simulink model "rfsoc4x2_ospfb_128"  (R2021a)
settings: Solver=VariableStepAuto  StartTime=0.0  StopTime=2048  RelTol=1e-3
undefined symbols (not defined in the file): pfb_coeff_gen_calc
libraries: xbsIndex_r4 x25898, casper_library_delays x113, casper_library_misc x68, xps_library x1
(part 49 of 221)

== system rfsoc4x2_ospfb_128/pfb_fir_real7/pol1_in1_first_tap2/delay_bram ==
  din : Inport
  constant : xbsIndex_r4/Constant  const=1  gui_display_data_type=Fixed-point  arith_type=Boolean  n_bits=16  bin_pt=14  preci_type=Single  exp_width=8  frac_width=24  explicit_period=on  period=1  equ=P=C  opselect=C  inp2=PCIN>>17  opr=+  inp1=P  carry=CIN  dbl_ovrd=off  block_type=constant
  counter : xbsIndex_r4/Counter  cnt_type=Count Limited  cnt_to=DelayLen - bram_latency - 1  operation=Up  start_count=0  cnt_by_val=1  arith_type=Unsigned  n_bits=4  bin_pt=0  load_pin=off  rst=off  en=off  explicit_period=on  period=1  use_behavioral_HDL=on  implementation=Fabric  use_rpm=off  dbl_ovrd=off  block_type=counter
  ram : xbsIndex_r4/Single Port RAM  depth=16  initVector=0  distributed_mem=Block RAM  write_mode=Read Before Write  rst=off  init_reg=0  en=off  optimize_latency=off  latency=bram_latency  optimize=Area  dbl_ovrd=off  simulation_type=fast_sim  block_type=spram
  dout : Outport  VectorParamsAs1DForOutWhenUnconnected=off
  wires:
  ram/1 -> dout/1
  constant/1 -> ram/3
  din/1 -> ram/2
  counter/1 -> ram/1

== system rfsoc4x2_ospfb_128/pfb_fir_real7/pol1_in1_first_tap3/delay_bram ==
  din : Inport
  constant : xbsIndex_r4/Constant  const=1  gui_display_data_type=Fixed-point  arith_type=Boolean  n_bits=16  bin_pt=14  preci_type=Single  exp_width=8  frac_width=24  explicit_period=on  period=1  equ=P=C  opselect=C  inp2=PCIN>>17  opr=+  inp1=P  carry=CIN  dbl_ovrd=off  block_type=constant
  counter : xbsIndex_r4/Counter  cnt_type=Count Limited  cnt_to=DelayLen - bram_latency - 1  operation=Up  start_count=0  cnt_by_val=1  arith_type=Unsigned  n_bits=4  bin_pt=0  load_pin=off  rst=off  en=off  explicit_period=on  period=1  use_behavioral_HDL=on  implementation=Fabric  use_rpm=off  dbl_ovrd=off  block_type=counter
  ram : xbsIndex_r4/Single Port RAM  depth=16  initVector=0  distributed_mem=Block RAM  write_mode=Read Before Write  rst=off  init_reg=0  en=off  optimize_latency=off  latency=bram_latency  optimize=Area  dbl_ovrd=off  simulation_type=fast_sim  block_type=spram
  dout : Outport  VectorParamsAs1DForOutWhenUnconnected=off
  wires:
  ram/1 -> dout/1
  constant/1 -> ram/3
  din/1 -> ram/2
  counter/1 -> ram/1

== system rfsoc4x2_ospfb_128/pfb_fir_real7/pol1_in1_first_tap4/delay_bram ==
  din : Inport
  constant : xbsIndex_r4/Constant  const=1  gui_display_data_type=Fixed-point  arith_type=Boolean  n_bits=16  bin_pt=14  preci_type=Single  exp_width=8  frac_width=24  explicit_period=on  period=1  equ=P=C  opselect=C  inp2=PCIN>>17  opr=+  inp1=P  carry=CIN  dbl_ovrd=off  block_type=constant
  counter : xbsIndex_r4/Counter  cnt_type=Count Limited  cnt_to=DelayLen - bram_latency - 1  operation=Up  start_count=0  cnt_by_val=1  arith_type=Unsigned  n_bits=4  bin_pt=0  load_pin=off  rst=off  en=off  explicit_period=on  period=1  use_behavioral_HDL=on  implementation=Fabric  use_rpm=off  dbl_ovrd=off  block_type=counter
  ram : xbsIndex_r4/Single Port RAM  depth=16  initVector=0  distributed_mem=Block RAM  write_mode=Read Before Write  rst=off  init_reg=0  en=off  optimize_latency=off  latency=bram_latency  optimize=Area  dbl_ovrd=off  simulation_type=fast_sim  block_type=spram
  dout : Outport  VectorParamsAs1DForOutWhenUnconnected=off
  wires:
  ram/1 -> dout/1
  constant/1 -> ram/3
  din/1 -> ram/2
  counter/1 -> ram/1

== system rfsoc4x2_ospfb_128/pfb_fir_real7/pol1_in1_first_tap5/delay_bram ==
  din : Inport
  constant : xbsIndex_r4/Constant  const=1  gui_display_data_type=Fixed-point  arith_type=Boolean  n_bits=16  bin_pt=14  preci_type=Single  exp_width=8  frac_width=24  explicit_period=on  period=1  equ=P=C  opselect=C  inp2=PCIN>>17  opr=+  inp1=P  carry=CIN  dbl_ovrd=off  block_type=constant
  counter : xbsIndex_r4/Counter  cnt_type=Count Limited  cnt_to=DelayLen - bram_latency - 1  operation=Up  start_count=0  cnt_by_val=1  arith_type=Unsigned  n_bits=4  bin_pt=0  load_pin=off  rst=off  en=off  explicit_period=on  period=1  use_behavioral_HDL=on  implementation=Fabric  use_rpm=off  dbl_ovrd=off  block_type=counter
  ram : xbsIndex_r4/Single Port RAM  depth=16  initVector=0  distributed_mem=Block RAM  write_mode=Read Before Write  rst=off  init_reg=0  en=off  optimize_latency=off  latency=bram_latency  optimize=Area  dbl_ovrd=off  simulation_type=fast_sim  block_type=spram
  dout : Outport  VectorParamsAs1DForOutWhenUnconnected=off
  wires:
  ram/1 -> dout/1
  constant/1 -> ram/3
  din/1 -> ram/2
  counter/1 -> ram/1

== system rfsoc4x2_ospfb_128/pfb_fir_real7/pol1_in1_first_tap6/delay_bram ==
  din : Inport
  constant : xbsIndex_r4/Constant  const=1  gui_display_data_type=Fixed-point  arith_type=Boolean  n_bits=16  bin_pt=14  preci_type=Single  exp_width=8  frac_width=24  explicit_period=on  period=1  equ=P=C  opselect=C  inp2=PCIN>>17  opr=+  inp1=P  carry=CIN  dbl_ovrd=off  block_type=constant
  counter : xbsIndex_r4/Counter  cnt_type=Count Limited  cnt_to=DelayLen - bram_latency - 1  operation=Up  start_count=0  cnt_by_val=1  arith_type=Unsigned  n_bits=4  bin_pt=0  load_pin=off  rst=off  en=off  explicit_period=on  period=1  use_behavioral_HDL=on  implementation=Fabric  use_rpm=off  dbl_ovrd=off  block_type=counter
  ram : xbsIndex_r4/Single Port RAM  depth=16  initVector=0  distributed_mem=Block RAM  write_mode=Read Before Write  rst=off  init_reg=0  en=off  optimize_latency=off  latency=bram_latency  optimize=Area  dbl_ovrd=off  simulation_type=fast_sim  block_type=spram
  dout : Outport  VectorParamsAs1DForOutWhenUnconnected=off
  wires:
  ram/1 -> dout/1
  constant/1 -> ram/3
  din/1 -> ram/2
  counter/1 -> ram/1

== system rfsoc4x2_ospfb_128/pfb_fir_real7/pol1_in1_first_tap7/delay_bram ==
  din : Inport
  constant : xbsIndex_r4/Constant  const=1  gui_display_data_type=Fixed-point  arith_type=Boolean  n_bits=16  bin_pt=14  preci_type=Single  exp_width=8  frac_width=24  explicit_period=on  period=1  equ=P=C  opselect=C  inp2=PCIN>>17  opr=+  inp1=P  carry=CIN  dbl_ovrd=off  block_type=constant
  counter : xbsIndex_r4/Counter  cnt_type=Count Limited  cnt_to=DelayLen - bram_latency - 1  operation=Up  start_count=0  cnt_by_val=1  arith_type=Unsigned  n_bits=4  bin_pt=0  load_pin=off  rst=off  en=off  explicit_period=on  period=1  use_behavioral_HDL=on  implementation=Fabric  use_rpm=off  dbl_ovrd=off  block_type=counter
  ram : xbsIndex_r4/Single Port RAM  depth=16  initVector=0  distributed_mem=Block RAM  write_mode=Read Before Write  rst=off  init_reg=0  en=off  optimize_latency=off  latency=bram_latency  optimize=Area  dbl_ovrd=off  simulation_type=fast_sim  block_type=spram
  dout : Outport  VectorParamsAs1DForOutWhenUnconnected=off
  wires:
  ram/1 -> dout/1
  constant/1 -> ram/3
  din/1 -> ram/2
  counter/1 -> ram/1

== system rfsoc4x2_ospfb_128/pfb_fir_real7/pol1_in1_first_tap8/delay_bram ==
  din : Inport
  constant : xbsIndex_r4/Constant  const=1  gui_display_data_type=Fixed-point  arith_type=Boolean  n_bits=16  bin_pt=14  preci_type=Single  exp_width=8  frac_width=24  explicit_period=on  period=1  equ=P=C  opselect=C  inp2=PCIN>>17  opr=+  inp1=P  carry=CIN  dbl_ovrd=off  block_type=constant
  counter : xbsIndex_r4/Counter  cnt_type=Count Limited  cnt_to=DelayLen - bram_latency - 1  operation=Up  start_count=0  cnt_by_val=1  arith_type=Unsigned  n_bits=4  bin_pt=0  load_pin=off  rst=off  en=off  explicit_period=on  period=1  use_behavioral_HDL=on  implementation=Fabric  use_rpm=off  dbl_ovrd=off  block_type=counter
  ram : xbsIndex_r4/Single Port RAM  depth=16  initVector=0  distributed_mem=Block RAM  write_mode=Read Before Write  rst=off  init_reg=0  en=off  optimize_latency=off  latency=bram_latency  optimize=Area  dbl_ovrd=off  simulation_type=fast_sim  block_type=spram
  dout : Outport  VectorParamsAs1DForOutWhenUnconnected=off
  wires:
  ram/1 -> dout/1
  constant/1 -> ram/3
  din/1 -> ram/2
  counter/1 -> ram/1

== system rfsoc4x2_ospfb_128/pfb_fir_real7/pol1_in1_first_tap9/delay_bram ==
  din : Inport
  constant : xbsIndex_r4/Constant  const=1  gui_display_data_type=Fixed-point  arith_type=Boolean  n_bits=16  bin_pt=14  preci_type=Single  exp_width=8  frac_width=24  explicit_period=on  period=1  equ=P=C  opselect=C  inp2=PCIN>>17  opr=+  inp1=P  carry=CIN  dbl_ovrd=off  block_type=constant
  counter : xbsIndex_r4/Counter  cnt_type=Count Limited  cnt_to=DelayLen - bram_latency - 1  operation=Up  start_count=0  cnt_by_val=1  arith_type=Unsigned  n_bits=4  bin_pt=0  load_pin=off  rst=off  en=off  explicit_period=on  period=1  use_behavioral_HDL=on  implementation=Fabric  use_rpm=off  dbl_ovrd=off  block_type=counter
  ram : xbsIndex_r4/Single Port RAM  depth=16  initVector=0  distributed_mem=Block RAM  write_mode=Read Before Write  rst=off  init_reg=0  en=off  optimize_latency=off  latency=bram_latency  optimize=Area  dbl_ovrd=off  simulation_type=fast_sim  block_type=spram
  dout : Outport  VectorParamsAs1DForOutWhenUnconnected=off
  wires:
  ram/1 -> dout/1
  constant/1 -> ram/3
  din/1 -> ram/2
  counter/1 -> ram/1

== system rfsoc4x2_ospfb_128/pfb_fir_real7/pol1_in1_tap1/delay_bram ==
  din : Inport
  constant : xbsIndex_r4/Constant  const=1  gui_display_data_type=Fixed-point  arith_type=Boolean  n_bits=16  bin_pt=14  preci_type=Single  exp_width=8  frac_width=24  explicit_period=on  period=1  equ=P=C  opselect=C  inp2=PCIN>>17  opr=+  inp1=P  carry=CIN  dbl_ovrd=off  block_type=constant
  counter : xbsIndex_r4/Counter  cnt_type=Count Limited  cnt_to=DelayLen - bram_latency - 1  operation=Up  start_count=0  cnt_by_val=1  arith_type=Unsigned  n_bits=4  bin_pt=0  load_pin=off  rst=off  en=off  explicit_period=on  period=1  use_behavioral_HDL=on  implementation=Fabric  use_rpm=off  dbl_ovrd=off  block_type=counter
  ram : xbsIndex_r4/Single Port RAM  depth=16  initVector=0  distributed_mem=Block RAM  write_mode=Read Before Write  rst=off  init_reg=0  en=off  optimize_latency=off  latency=bram_latency  optimize=Area  dbl_ovrd=off  simulation_type=fast_sim  block_type=spram
  dout : Outport  VectorParamsAs1DForOutWhenUnconnected=off
  wires:
  ram/1 -> dout/1
  constant/1 -> ram/3
  din/1 -> ram/2
  counter/1 -> ram/1

== system rfsoc4x2_ospfb_128/pfb_fir_real7/pol1_in1_tap10/delay_bram ==
  din : Inport
  constant : xbsIndex_r4/Constant  const=1  gui_display_data_type=Fixed-point  arith_type=Boolean  n_bits=16  bin_pt=14  preci_type=Single  exp_width=8  frac_width=24  explicit_period=on  period=1  equ=P=C  opselect=C  inp2=PCIN>>17  opr=+  inp1=P  carry=CIN  dbl_ovrd=off  block_type=constant
  counter : xbsIndex_r4/Counter  cnt_type=Count Limited  cnt_to=DelayLen - bram_latency - 1  operation=Up  start_count=0  cnt_by_val=1  arith_type=Unsigned  n_bits=4  bin_pt=0  load_pin=off  rst=off  en=off  explicit_period=on  period=1  use_behavioral_HDL=on  implementation=Fabric  use_rpm=off  dbl_ovrd=off  block_type=counter
  ram : xbsIndex_r4/Single Port RAM  depth=16  initVector=0  distributed_mem=Block RAM  write_mode=Read Before Write  rst=off  init_reg=0  en=off  optimize_latency=off  latency=bram_latency  optimize=Area  dbl_ovrd=off  simulation_type=fast_sim  block_type=spram
  dout : Outport  VectorParamsAs1DForOutWhenUnconnected=off
  wires:
  ram/1 -> dout/1
  constant/1 -> ram/3
  din/1 -> ram/2
  counter/1 -> ram/1

== system rfsoc4x2_ospfb_128/pfb_fir_real7/pol1_in1_tap11/delay_bram ==
  din : Inport
  constant : xbsIndex_r4/Constant  const=1  gui_display_data_type=Fixed-point  arith_type=Boolean  n_bits=16  bin_pt=14  preci_type=Single  exp_width=8  frac_width=24  explicit_period=on  period=1  equ=P=C  opselect=C  inp2=PCIN>>17  opr=+  inp1=P  carry=CIN  dbl_ovrd=off  block_type=constant
  counter : xbsIndex_r4/Counter  cnt_type=Count Limited  cnt_to=DelayLen - bram_latency - 1  operation=Up  start_count=0  cnt_by_val=1  arith_type=Unsigned  n_bits=4  bin_pt=0  load_pin=off  rst=off  en=off  explicit_period=on  period=1  use_behavioral_HDL=on  implementation=Fabric  use_rpm=off  dbl_ovrd=off  block_type=counter
  ram : xbsIndex_r4/Single Port RAM  depth=16  initVector=0  distributed_mem=Block RAM  write_mode=Read Before Write  rst=off  init_reg=0  en=off  optimize_latency=off  latency=bram_latency  optimize=Area  dbl_ovrd=off  simulation_type=fast_sim  block_type=spram
  dout : Outport  VectorParamsAs1DForOutWhenUnconnected=off
  wires:
  ram/1 -> dout/1
  constant/1 -> ram/3
  din/1 -> ram/2
  counter/1 -> ram/1

== system rfsoc4x2_ospfb_128/pfb_fir_real7/pol1_in1_tap12/delay_bram ==
  din : Inport
  constant : xbsIndex_r4/Constant  const=1  gui_display_data_type=Fixed-point  arith_type=Boolean  n_bits=16  bin_pt=14  preci_type=Single  exp_width=8  frac_width=24  explicit_period=on  period=1  equ=P=C  opselect=C  inp2=PCIN>>17  opr=+  inp1=P  carry=CIN  dbl_ovrd=off  block_type=constant
  counter : xbsIndex_r4/Counter  cnt_type=Count Limited  cnt_to=DelayLen - bram_latency - 1  operation=Up  start_count=0  cnt_by_val=1  arith_type=Unsigned  n_bits=4  bin_pt=0  load_pin=off  rst=off  en=off  explicit_period=on  period=1  use_behavioral_HDL=on  implementation=Fabric  use_rpm=off  dbl_ovrd=off  block_type=counter
  ram : xbsIndex_r4/Single Port RAM  depth=16  initVector=0  distributed_mem=Block RAM  write_mode=Read Before Write  rst=off  init_reg=0  en=off  optimize_latency=off  latency=bram_latency  optimize=Area  dbl_ovrd=off  simulation_type=fast_sim  block_type=spram
  dout : Outport  VectorParamsAs1DForOutWhenUnconnected=off
  wires:
  ram/1 -> dout/1
  constant/1 -> ram/3
  din/1 -> ram/2
  counter/1 -> ram/1

== system rfsoc4x2_ospfb_128/pfb_fir_real7/pol1_in1_tap13/delay_bram ==
  din : Inport
  constant : xbsIndex_r4/Constant  const=1  gui_display_data_type=Fixed-point  arith_type=Boolean  n_bits=16  bin_pt=14  preci_type=Single  exp_width=8  frac_width=24  explicit_period=on  period=1  equ=P=C  opselect=C  inp2=PCIN>>17  opr=+  inp1=P  carry=CIN  dbl_ovrd=off  block_type=constant
  counter : xbsIndex_r4/Counter  cnt_type=Count Limited  cnt_to=DelayLen - bram_latency - 1  operation=Up  start_count=0  cnt_by_val=1  arith_type=Unsigned  n_bits=4  bin_pt=0  load_pin=off  rst=off  en=off  explicit_period=on  period=1  use_behavioral_HDL=on  implementation=Fabric  use_rpm=off  dbl_ovrd=off  block_type=counter
  ram : xbsIndex_r4/Single Port RAM  depth=16  initVector=0  distributed_mem=Block RAM  write_mode=Read Before Write  rst=off  init_reg=0  en=off  optimize_latency=off  latency=bram_latency  optimize=Area  dbl_ovrd=off  simulation_type=fast_sim  block_type=spram
  dout : Outport  VectorParamsAs1DForOutWhenUnconnected=off
  wires:
  ram/1 -> dout/1
  constant/1 -> ram/3
  din/1 -> ram/2
  counter/1 -> ram/1

== system rfsoc4x2_ospfb_128/pfb_fir_real7/pol1_in1_tap14/delay_bram ==
  din : Inport
  constant : xbsIndex_r4/Constant  const=1  gui_display_data_type=Fixed-point  arith_type=Boolean  n_bits=16  bin_pt=14  preci_type=Single  exp_width=8  frac_width=24  explicit_period=on  period=1  equ=P=C  opselect=C  inp2=PCIN>>17  opr=+  inp1=P  carry=CIN  dbl_ovrd=off  block_type=constant
  counter : xbsIndex_r4/Counter  cnt_type=Count Limited  cnt_to=DelayLen - bram_latency - 1  operation=Up  start_count=0  cnt_by_val=1  arith_type=Unsigned  n_bits=4  bin_pt=0  load_pin=off  rst=off  en=off  explicit_period=on  period=1  use_behavioral_HDL=on  implementation=Fabric  use_rpm=off  dbl_ovrd=off  block_type=counter
  ram : xbsIndex_r4/Single Port RAM  depth=16  initVector=0  distributed_mem=Block RAM  write_mode=Read Before Write  rst=off  init_reg=0  en=off  optimize_latency=off  latency=bram_latency  optimize=Area  dbl_ovrd=off  simulation_type=fast_sim  block_type=spram
  dout : Outport  VectorParamsAs1DForOutWhenUnconnected=off
  wires:
  ram/1 -> dout/1
  constant/1 -> ram/3
  din/1 -> ram/2
  counter/1 -> ram/1

== system rfsoc4x2_ospfb_128/pfb_fir_real7/pol1_in1_tap15/delay_bram ==
  din : Inport
  constant : xbsIndex_r4/Constant  const=1  gui_display_data_type=Fixed-point  arith_type=Boolean  n_bits=16  bin_pt=14  preci_type=Single  exp_width=8  frac_width=24  explicit_period=on  period=1  equ=P=C  opselect=C  inp2=PCIN>>17  opr=+  inp1=P  carry=CIN  dbl_ovrd=off  block_type=constant
  counter : xbsIndex_r4/Counter  cnt_type=Count Limited  cnt_to=DelayLen - bram_latency - 1  operation=Up  start_count=0  cnt_by_val=1  arith_type=Unsigned  n_bits=4  bin_pt=0  load_pin=off  rst=off  en=off  explicit_period=on  period=1  use_behavioral_HDL=on  implementation=Fabric  use_rpm=off  dbl_ovrd=off  block_type=counter
  ram : xbsIndex_r4/Single Port RAM  depth=16  initVector=0  distributed_mem=Block RAM  write_mode=Read Before Write  rst=off  init_reg=0  en=off  optimize_latency=off  latency=bram_latency  optimize=Area  dbl_ovrd=off  simulation_type=fast_sim  block_type=spram
  dout : Outport  VectorParamsAs1DForOutWhenUnconnected=off
  wires:
  ram/1 -> dout/1
  constant/1 -> ram/3
  din/1 -> ram/2
  counter/1 -> ram/1

== system rfsoc4x2_ospfb_128/pfb_fir_real7/pol1_in1_tap16/delay_bram ==
  din : Inport
  constant : xbsIndex_r4/Constant  const=1  gui_display_data_type=Fixed-point  arith_type=Boolean  n_bits=16  bin_pt=14  preci_type=Single  exp_width=8  frac_width=24  explicit_period=on  period=1  equ=P=C  opselect=C  inp2=PCIN>>17  opr=+  inp1=P  carry=CIN  dbl_ovrd=off  block_type=constant
  counter : xbsIndex_r4/Counter  cnt_type=Count Limited  cnt_to=DelayLen - bram_latency - 1  operation=Up  start_count=0  cnt_by_val=1  arith_type=Unsigned  n_bits=4  bin_pt=0  load_pin=off  rst=off  en=off  explicit_period=on  period=1  use_behavioral_HDL=on  implementation=Fabric  use_rpm=off  dbl_ovrd=off  block_type=counter
  ram : xbsIndex_r4/Single Port RAM  depth=16  initVector=0  distributed_mem=Block RAM  write_mode=Read Before Write  rst=off  init_reg=0  en=off  optimize_latency=off  latency=bram_latency  optimize=Area  dbl_ovrd=off  simulation_type=fast_sim  block_type=spram
  dout : Outport  VectorParamsAs1DForOutWhenUnconnected=off
  wires:
  ram/1 -> dout/1
  constant/1 -> ram/3
  din/1 -> ram/2
  counter/1 -> ram/1

== system rfsoc4x2_ospfb_128/pfb_fir_real7/pol1_in1_tap17/delay_bram ==
  din : Inport
  constant : xbsIndex_r4/Constant  const=1  gui_display_data_type=Fixed-point  arith_type=Boolean  n_bits=16  bin_pt=14  preci_type=Single  exp_width=8  frac_width=24  explicit_period=on  period=1  equ=P=C  opselect=C  inp2=PCIN>>17  opr=+  inp1=P  carry=CIN  dbl_ovrd=off  block_type=constant
  counter : xbsIndex_r4/Counter  cnt_type=Count Limited  cnt_to=DelayLen - bram_latency - 1  operation=Up  start_count=0  cnt_by_val=1  arith_type=Unsigned  n_bits=4  bin_pt=0  load_pin=off  rst=off  en=off  explicit_period=on  period=1  use_behavioral_HDL=on  implementation=Fabric  use_rpm=off  dbl_ovrd=off  block_type=counter
  ram : xbsIndex_r4/Single Port RAM  depth=16  initVector=0  distributed_mem=Block RAM  write_mode=Read Before Write  rst=off  init_reg=0  en=off  optimize_latency=off  latency=bram_latency  optimize=Area  dbl_ovrd=off  simulation_type=fast_sim  block_type=spram
  dout : Outport  VectorParamsAs1DForOutWhenUnconnected=off
  wires:
  ram/1 -> dout/1
  constant/1 -> ram/3
  din/1 -> ram/2
  counter/1 -> ram/1

== system rfsoc4x2_ospfb_128/pfb_fir_real7/pol1_in1_tap18/delay_bram ==
  din : Inport
  constant : xbsIndex_r4/Constant  const=1  gui_display_data_type=Fixed-point  arith_type=Boolean  n_bits=16  bin_pt=14  preci_type=Single  exp_width=8  frac_width=24  explicit_period=on  period=1  equ=P=C  opselect=C  inp2=PCIN>>17  opr=+  inp1=P  carry=CIN  dbl_ovrd=off  block_type=constant
  counter : xbsIndex_r4/Counter  cnt_type=Count Limited  cnt_to=DelayLen - bram_latency - 1  operation=Up  start_count=0  cnt_by_val=1  arith_type=Unsigned  n_bits=4  bin_pt=0  load_pin=off  rst=off  en=off  explicit_period=on  period=1  use_behavioral_HDL=on  implementation=Fabric  use_rpm=off  dbl_ovrd=off  block_type=counter
  ram : xbsIndex_r4/Single Port RAM  depth=16  initVector=0  distributed_mem=Block RAM  write_mode=Read Before Write  rst=off  init_reg=0  en=off  optimize_latency=off  latency=bram_latency  optimize=Area  dbl_ovrd=off  simulation_type=fast_sim  block_type=spram
  dout : Outport  VectorParamsAs1DForOutWhenUnconnected=off
  wires:
  ram/1 -> dout/1
  constant/1 -> ram/3
  din/1 -> ram/2
  counter/1 -> ram/1

== system rfsoc4x2_ospfb_128/pfb_fir_real7/pol1_in1_tap19/delay_bram ==
  din : Inport
  constant : xbsIndex_r4/Constant  const=1  gui_display_data_type=Fixed-point  arith_type=Boolean  n_bits=16  bin_pt=14  preci_type=Single  exp_width=8  frac_width=24  explicit_period=on  period=1  equ=P=C  opselect=C  inp2=PCIN>>17  opr=+  inp1=P  carry=CIN  dbl_ovrd=off  block_type=constant
  counter : xbsIndex_r4/Counter  cnt_type=Count Limited  cnt_to=DelayLen - bram_latency - 1  operation=Up  start_count=0  cnt_by_val=1  arith_type=Unsigned  n_bits=4  bin_pt=0  load_pin=off  rst=off  en=off  explicit_period=on  period=1  use_behavioral_HDL=on  implementation=Fabric  use_rpm=off  dbl_ovrd=off  block_type=counter
  ram : xbsIndex_r4/Single Port RAM  depth=16  initVector=0  distributed_mem=Block RAM  write_mode=Read Before Write  rst=off  init_reg=0  en=off  optimize_latency=off  latency=bram_latency  optimize=Area  dbl_ovrd=off  simulation_type=fast_sim  block_type=spram
  dout : Outport  VectorParamsAs1DForOutWhenUnconnected=off
  wires:
  ram/1 -> dout/1
  constant/1 -> ram/3
  din/1 -> ram/2
  counter/1 -> ram/1

== system rfsoc4x2_ospfb_128/pfb_fir_real7/pol1_in1_tap2/delay_bram ==
  din : Inport
  constant : xbsIndex_r4/Constant  const=1  gui_display_data_type=Fixed-point  arith_type=Boolean  n_bits=16  bin_pt=14  preci_type=Single  exp_width=8  frac_width=24  explicit_period=on  period=1  equ=P=C  opselect=C  inp2=PCIN>>17  opr=+  inp1=P  carry=CIN  dbl_ovrd=off  block_type=constant
  counter : xbsIndex_r4/Counter  cnt_type=Count Limited  cnt_to=DelayLen - bram_latency - 1  operation=Up  start_count=0  cnt_by_val=1  arith_type=Unsigned  n_bits=4  bin_pt=0  load_pin=off  rst=off  en=off  explicit_period=on  period=1  use_behavioral_HDL=on  implementation=Fabric  use_rpm=off  dbl_ovrd=off  block_type=counter
  ram : xbsIndex_r4/Single Port RAM  depth=16  initVector=0  distributed_mem=Block RAM  write_mode=Read Before Write  rst=off  init_reg=0  en=off  optimize_latency=off  latency=bram_latency  optimize=Area  dbl_ovrd=off  simulation_type=fast_sim  block_type=spram
  dout : Outport  VectorParamsAs1DForOutWhenUnconnected=off
  wires:
  ram/1 -> dout/1
  constant/1 -> ram/3
  din/1 -> ram/2
  counter/1 -> ram/1

== system rfsoc4x2_ospfb_128/pfb_fir_real7/pol1_in1_tap20/delay_bram ==
  din : Inport
  constant : xbsIndex_r4/Constant  const=1  gui_display_data_type=Fixed-point  arith_type=Boolean  n_bits=16  bin_pt=14  preci_type=Single  exp_width=8  frac_width=24  explicit_period=on  period=1  equ=P=C  opselect=C  inp2=PCIN>>17  opr=+  inp1=P  carry=CIN  dbl_ovrd=off  block_type=constant
  counter : xbsIndex_r4/Counter  cnt_type=Count Limited  cnt_to=DelayLen - bram_latency - 1  operation=Up  start_count=0  cnt_by_val=1  arith_type=Unsigned  n_bits=4  bin_pt=0  load_pin=off  rst=off  en=off  explicit_period=on  period=1  use_behavioral_HDL=on  implementation=Fabric  use_rpm=off  dbl_ovrd=off  block_type=counter
  ram : xbsIndex_r4/Single Port RAM  depth=16  initVector=0  distributed_mem=Block RAM  write_mode=Read Before Write  rst=off  init_reg=0  en=off  optimize_latency=off  latency=bram_latency  optimize=Area  dbl_ovrd=off  simulation_type=fast_sim  block_type=spram
  dout : Outport  VectorParamsAs1DForOutWhenUnconnected=off
  wires:
  ram/1 -> dout/1
  constant/1 -> ram/3
  din/1 -> ram/2
  counter/1 -> ram/1

== system rfsoc4x2_ospfb_128/pfb_fir_real7/pol1_in1_tap21/delay_bram ==
  din : Inport
  constant : xbsIndex_r4/Constant  const=1  gui_display_data_type=Fixed-point  arith_type=Boolean  n_bits=16  bin_pt=14  preci_type=Single  exp_width=8  frac_width=24  explicit_period=on  period=1  equ=P=C  opselect=C  inp2=PCIN>>17  opr=+  inp1=P  carry=CIN  dbl_ovrd=off  block_type=constant
  counter : xbsIndex_r4/Counter  cnt_type=Count Limited  cnt_to=DelayLen - bram_latency - 1  operation=Up  start_count=0  cnt_by_val=1  arith_type=Unsigned  n_bits=4  bin_pt=0  load_pin=off  rst=off  en=off  explicit_period=on  period=1  use_behavioral_HDL=on  implementation=Fabric  use_rpm=off  dbl_ovrd=off  block_type=counter
  ram : xbsIndex_r4/Single Port RAM  depth=16  initVector=0  distributed_mem=Block RAM  write_mode=Read Before Write  rst=off  init_reg=0  en=off  optimize_latency=off  latency=bram_latency  optimize=Area  dbl_ovrd=off  simulation_type=fast_sim  block_type=spram
  dout : Outport  VectorParamsAs1DForOutWhenUnconnected=off
  wires:
  ram/1 -> dout/1
  constant/1 -> ram/3
  din/1 -> ram/2
  counter/1 -> ram/1

== system rfsoc4x2_ospfb_128/pfb_fir_real7/pol1_in1_tap22/delay_bram ==
  din : Inport
  constant : xbsIndex_r4/Constant  const=1  gui_display_data_type=Fixed-point  arith_type=Boolean  n_bits=16  bin_pt=14  preci_type=Single  exp_width=8  frac_width=24  explicit_period=on  period=1  equ=P=C  opselect=C  inp2=PCIN>>17  opr=+  inp1=P  carry=CIN  dbl_ovrd=off  block_type=constant
  counter : xbsIndex_r4/Counter  cnt_type=Count Limited  cnt_to=DelayLen - bram_latency - 1  operation=Up  start_count=0  cnt_by_val=1  arith_type=Unsigned  n_bits=4  bin_pt=0  load_pin=off  rst=off  en=off  explicit_period=on  period=1  use_behavioral_HDL=on  implementation=Fabric  use_rpm=off  dbl_ovrd=off  block_type=counter
  ram : xbsIndex_r4/Single Port RAM  depth=16  initVector=0  distributed_mem=Block RAM  write_mode=Read Before Write  rst=off  init_reg=0  en=off  optimize_latency=off  latency=bram_latency  optimize=Area  dbl_ovrd=off  simulation_type=fast_sim  block_type=spram
  dout : Outport  VectorParamsAs1DForOutWhenUnconnected=off
  wires:
  ram/1 -> dout/1
  constant/1 -> ram/3
  din/1 -> ram/2
  counter/1 -> ram/1

== system rfsoc4x2_ospfb_128/pfb_fir_real7/pol1_in1_tap23/delay_bram ==
  din : Inport
  constant : xbsIndex_r4/Constant  const=1  gui_display_data_type=Fixed-point  arith_type=Boolean  n_bits=16  bin_pt=14  preci_type=Single  exp_width=8  frac_width=24  explicit_period=on  period=1  equ=P=C  opselect=C  inp2=PCIN>>17  opr=+  inp1=P  carry=CIN  dbl_ovrd=off  block_type=constant
  counter : xbsIndex_r4/Counter  cnt_type=Count Limited  cnt_to=DelayLen - bram_latency - 1  operation=Up  start_count=0  cnt_by_val=1  arith_type=Unsigned  n_bits=4  bin_pt=0  load_pin=off  rst=off  en=off  explicit_period=on  period=1  use_behavioral_HDL=on  implementation=Fabric  use_rpm=off  dbl_ovrd=off  block_type=counter
  ram : xbsIndex_r4/Single Port RAM  depth=16  initVector=0  distributed_mem=Block RAM  write_mode=Read Before Write  rst=off  init_reg=0  en=off  optimize_latency=off  latency=bram_latency  optimize=Area  dbl_ovrd=off  simulation_type=fast_sim  block_type=spram
  dout : Outport  VectorParamsAs1DForOutWhenUnconnected=off
  wires:
  ram/1 -> dout/1
  constant/1 -> ram/3
  din/1 -> ram/2
  counter/1 -> ram/1

== system rfsoc4x2_ospfb_128/pfb_fir_real7/pol1_in1_tap24/delay_bram ==
  din : Inport
  constant : xbsIndex_r4/Constant  const=1  gui_display_data_type=Fixed-point  arith_type=Boolean  n_bits=16  bin_pt=14  preci_type=Single  exp_width=8  frac_width=24  explicit_period=on  period=1  equ=P=C  opselect=C  inp2=PCIN>>17  opr=+  inp1=P  carry=CIN  dbl_ovrd=off  block_type=constant
  counter : xbsIndex_r4/Counter  cnt_type=Count Limited  cnt_to=DelayLen - bram_latency - 1  operation=Up  start_count=0  cnt_by_val=1  arith_type=Unsigned  n_bits=4  bin_pt=0  load_pin=off  rst=off  en=off  explicit_period=on  period=1  use_behavioral_HDL=on  implementation=Fabric  use_rpm=off  dbl_ovrd=off  block_type=counter
  ram : xbsIndex_r4/Single Port RAM  depth=16  initVector=0  distributed_mem=Block RAM  write_mode=Read Before Write  rst=off  init_reg=0  en=off  optimize_latency=off  latency=bram_latency  optimize=Area  dbl_ovrd=off  simulation_type=fast_sim  block_type=spram
  dout : Outport  VectorParamsAs1DForOutWhenUnconnected=off
  wires:
  ram/1 -> dout/1
  constant/1 -> ram/3
  din/1 -> ram/2
  counter/1 -> ram/1

== system rfsoc4x2_ospfb_128/pfb_fir_real7/pol1_in1_tap25/delay_bram ==
  din : Inport
  constant : xbsIndex_r4/Constant  const=1  gui_display_data_type=Fixed-point  arith_type=Boolean  n_bits=16  bin_pt=14  preci_type=Single  exp_width=8  frac_width=24  explicit_period=on  period=1  equ=P=C  opselect=C  inp2=PCIN>>17  opr=+  inp1=P  carry=CIN  dbl_ovrd=off  block_type=constant
  counter : xbsIndex_r4/Counter  cnt_type=Count Limited  cnt_to=DelayLen - bram_latency - 1  operation=Up  start_count=0  cnt_by_val=1  arith_type=Unsigned  n_bits=4  bin_pt=0  load_pin=off  rst=off  en=off  explicit_period=on  period=1  use_behavioral_HDL=on  implementation=Fabric  use_rpm=off  dbl_ovrd=off  block_type=counter
  ram : xbsIndex_r4/Single Port RAM  depth=16  initVector=0  distributed_mem=Block RAM  write_mode=Read Before Write  rst=off  init_reg=0  en=off  optimize_latency=off  latency=bram_latency  optimize=Area  dbl_ovrd=off  simulation_type=fast_sim  block_type=spram
  dout : Outport  VectorParamsAs1DForOutWhenUnconnected=off
  wires:
  ram/1 -> dout/1
  constant/1 -> ram/3
  din/1 -> ram/2
  counter/1 -> ram/1

== system rfsoc4x2_ospfb_128/pfb_fir_real7/pol1_in1_tap26/delay_bram ==
  din : Inport
  constant : xbsIndex_r4/Constant  const=1  gui_display_data_type=Fixed-point  arith_type=Boolean  n_bits=16  bin_pt=14  preci_type=Single  exp_width=8  frac_width=24  explicit_period=on  period=1  equ=P=C  opselect=C  inp2=PCIN>>17  opr=+  inp1=P  carry=CIN  dbl_ovrd=off  block_type=constant
  counter : xbsIndex_r4/Counter  cnt_type=Count Limited  cnt_to=DelayLen - bram_latency - 1  operation=Up  start_count=0  cnt_by_val=1  arith_type=Unsigned  n_bits=4  bin_pt=0  load_pin=off  rst=off  en=off  explicit_period=on  period=1  use_behavioral_HDL=on  implementation=Fabric  use_rpm=off  dbl_ovrd=off  block_type=counter
  ram : xbsIndex_r4/Single Port RAM  depth=16  initVector=0  distributed_mem=Block RAM  write_mode=Read Before Write  rst=off  init_reg=0  en=off  optimize_latency=off  latency=bram_latency  optimize=Area  dbl_ovrd=off  simulation_type=fast_sim  block_type=spram
  dout : Outport  VectorParamsAs1DForOutWhenUnconnected=off
  wires:
  ram/1 -> dout/1
  constant/1 -> ram/3
  din/1 -> ram/2
  counter/1 -> ram/1

== system rfsoc4x2_ospfb_128/pfb_fir_real7/pol1_in1_tap27/delay_bram ==
  din : Inport
  constant : xbsIndex_r4/Constant  const=1  gui_display_data_type=Fixed-point  arith_type=Boolean  n_bits=16  bin_pt=14  preci_type=Single  exp_width=8  frac_width=24  explicit_period=on  period=1  equ=P=C  opselect=C  inp2=PCIN>>17  opr=+  inp1=P  carry=CIN  dbl_ovrd=off  block_type=constant
  counter : xbsIndex_r4/Counter  cnt_type=Count Limited  cnt_to=DelayLen - bram_latency - 1  operation=Up  start_count=0  cnt_by_val=1  arith_type=Unsigned  n_bits=4  bin_pt=0  load_pin=off  rst=off  en=off  explicit_period=on  period=1  use_behavioral_HDL=on  implementation=Fabric  use_rpm=off  dbl_ovrd=off  block_type=counter
  ram : xbsIndex_r4/Single Port RAM  depth=16  initVector=0  distributed_mem=Block RAM  write_mode=Read Before Write  rst=off  init_reg=0  en=off  optimize_latency=off  latency=bram_latency  optimize=Area  dbl_ovrd=off  simulation_type=fast_sim  block_type=spram
  dout : Outport  VectorParamsAs1DForOutWhenUnconnected=off
  wires:
  ram/1 -> dout/1
  constant/1 -> ram/3
  din/1 -> ram/2
  counter/1 -> ram/1

== system rfsoc4x2_ospfb_128/pfb_fir_real7/pol1_in1_tap28/delay_bram ==
  din : Inport
  constant : xbsIndex_r4/Constant  const=1  gui_display_data_type=Fixed-point  arith_type=Boolean  n_bits=16  bin_pt=14  preci_type=Single  exp_width=8  frac_width=24  explicit_period=on  period=1  equ=P=C  opselect=C  inp2=PCIN>>17  opr=+  inp1=P  carry=CIN  dbl_ovrd=off  block_type=constant
  counter : xbsIndex_r4/Counter  cnt_type=Count Limited  cnt_to=DelayLen - bram_latency - 1  operation=Up  start_count=0  cnt_by_val=1  arith_type=Unsigned  n_bits=4  bin_pt=0  load_pin=off  rst=off  en=off  explicit_period=on  period=1  use_behavioral_HDL=on  implementation=Fabric  use_rpm=off  dbl_ovrd=off  block_type=counter
  ram : xbsIndex_r4/Single Port RAM  depth=16  initVector=0  distributed_mem=Block RAM  write_mode=Read Before Write  rst=off  init_reg=0  en=off  optimize_latency=off  latency=bram_latency  optimize=Area  dbl_ovrd=off  simulation_type=fast_sim  block_type=spram
  dout : Outport  VectorParamsAs1DForOutWhenUnconnected=off
  wires:
  ram/1 -> dout/1
  constant/1 -> ram/3
  din/1 -> ram/2
  counter/1 -> ram/1

== system rfsoc4x2_ospfb_128/pfb_fir_real7/pol1_in1_tap29/delay_bram ==
  din : Inport
  constant : xbsIndex_r4/Constant  const=1  gui_display_data_type=Fixed-point  arith_type=Boolean  n_bits=16  bin_pt=14  preci_type=Single  exp_width=8  frac_width=24  explicit_period=on  period=1  equ=P=C  opselect=C  inp2=PCIN>>17  opr=+  inp1=P  carry=CIN  dbl_ovrd=off  block_type=constant
  counter : xbsIndex_r4/Counter  cnt_type=Count Limited  cnt_to=DelayLen - bram_latency - 1  operation=Up  start_count=0  cnt_by_val=1  arith_type=Unsigned  n_bits=4  bin_pt=0  load_pin=off  rst=off  en=off  explicit_period=on  period=1  use_behavioral_HDL=on  implementation=Fabric  use_rpm=off  dbl_ovrd=off  block_type=counter
  ram : xbsIndex_r4/Single Port RAM  depth=16  initVector=0  distributed_mem=Block RAM  write_mode=Read Before Write  rst=off  init_reg=0  en=off  optimize_latency=off  latency=bram_latency  optimize=Area  dbl_ovrd=off  simulation_type=fast_sim  block_type=spram
  dout : Outport  VectorParamsAs1DForOutWhenUnconnected=off
  wires:
  ram/1 -> dout/1
  constant/1 -> ram/3
  din/1 -> ram/2
  counter/1 -> ram/1

== system rfsoc4x2_ospfb_128/pfb_fir_real7/pol1_in1_tap3/delay_bram ==
  din : Inport
  constant : xbsIndex_r4/Constant  const=1  gui_display_data_type=Fixed-point  arith_type=Boolean  n_bits=16  bin_pt=14  preci_type=Single  exp_width=8  frac_width=24  explicit_period=on  period=1  equ=P=C  opselect=C  inp2=PCIN>>17  opr=+  inp1=P  carry=CIN  dbl_ovrd=off  block_type=constant
  counter : xbsIndex_r4/Counter  cnt_type=Count Limited  cnt_to=DelayLen - bram_latency - 1  operation=Up  start_count=0  cnt_by_val=1  arith_type=Unsigned  n_bits=4  bin_pt=0  load_pin=off  rst=off  en=off  explicit_period=on  period=1  use_behavioral_HDL=on  implementation=Fabric  use_rpm=off  dbl_ovrd=off  block_type=counter
  ram : xbsIndex_r4/Single Port RAM  depth=16  initVector=0  distributed_mem=Block RAM  write_mode=Read Before Write  rst=off  init_reg=0  en=off  optimize_latency=off  latency=bram_latency  optimize=Area  dbl_ovrd=off  simulation_type=fast_sim  block_type=spram
  dout : Outport  VectorParamsAs1DForOutWhenUnconnected=off
  wires:
  ram/1 -> dout/1
  constant/1 -> ram/3
  din/1 -> ram/2
  counter/1 -> ram/1

== system rfsoc4x2_ospfb_128/pfb_fir_real7/pol1_in1_tap30/delay_bram ==
  din : Inport
  constant : xbsIndex_r4/Constant  const=1  gui_display_data_type=Fixed-point  arith_type=Boolean  n_bits=16  bin_pt=14  preci_type=Single  exp_width=8  frac_width=24  explicit_period=on  period=1  equ=P=C  opselect=C  inp2=PCIN>>17  opr=+  inp1=P  carry=CIN  dbl_ovrd=off  block_type=constant
  counter : xbsIndex_r4/Counter  cnt_type=Count Limited  cnt_to=DelayLen - bram_latency - 1  operation=Up  start_count=0  cnt_by_val=1  arith_type=Unsigned  n_bits=4  bin_pt=0  load_pin=off  rst=off  en=off  explicit_period=on  period=1  use_behavioral_HDL=on  implementation=Fabric  use_rpm=off  dbl_ovrd=off  block_type=counter
  ram : xbsIndex_r4/Single Port RAM  depth=16  initVector=0  distributed_mem=Block RAM  write_mode=Read Before Write  rst=off  init_reg=0  en=off  optimize_latency=off  latency=bram_latency  optimize=Area  dbl_ovrd=off  simulation_type=fast_sim  block_type=spram
  dout : Outport  VectorParamsAs1DForOutWhenUnconnected=off
  wires:
  ram/1 -> dout/1
  constant/1 -> ram/3
  din/1 -> ram/2
  counter/1 -> ram/1

== system rfsoc4x2_ospfb_128/pfb_fir_real7/pol1_in1_tap31/delay_bram ==
  din : Inport
  constant : xbsIndex_r4/Constant  const=1  gui_display_data_type=Fixed-point  arith_type=Boolean  n_bits=16  bin_pt=14  preci_type=Single  exp_width=8  frac_width=24  explicit_period=on  period=1  equ=P=C  opselect=C  inp2=PCIN>>17  opr=+  inp1=P  carry=CIN  dbl_ovrd=off  block_type=constant
  counter : xbsIndex_r4/Counter  cnt_type=Count Limited  cnt_to=DelayLen - bram_latency - 1  operation=Up  start_count=0  cnt_by_val=1  arith_type=Unsigned  n_bits=4  bin_pt=0  load_pin=off  rst=off  en=off  explicit_period=on  period=1  use_behavioral_HDL=on  implementation=Fabric  use_rpm=off  dbl_ovrd=off  block_type=counter
  ram : xbsIndex_r4/Single Port RAM  depth=16  initVector=0  distributed_mem=Block RAM  write_mode=Read Before Write  rst=off  init_reg=0  en=off  optimize_latency=off  latency=bram_latency  optimize=Area  dbl_ovrd=off  simulation_type=fast_sim  block_type=spram
  dout : Outport  VectorParamsAs1DForOutWhenUnconnected=off
  wires:
  ram/1 -> dout/1
  constant/1 -> ram/3
  din/1 -> ram/2
  counter/1 -> ram/1

== system rfsoc4x2_ospfb_128/pfb_fir_real7/pol1_in1_tap32/delay_bram ==
  din : Inport
  constant : xbsIndex_r4/Constant  const=1  gui_display_data_type=Fixed-point  arith_type=Boolean  n_bits=16  bin_pt=14  preci_type=Single  exp_width=8  frac_width=24  explicit_period=on  period=1  equ=P=C  opselect=C  inp2=PCIN>>17  opr=+  inp1=P  carry=CIN  dbl_ovrd=off  block_type=constant
  counter : xbsIndex_r4/Counter  cnt_type=Count Limited  cnt_to=DelayLen - bram_latency - 1  operation=Up  start_count=0  cnt_by_val=1  arith_type=Unsigned  n_bits=4  bin_pt=0  load_pin=off  rst=off  en=off  explicit_period=on  period=1  use_behavioral_HDL=on  implementation=Fabric  use_rpm=off  dbl_ovrd=off  block_type=counter
  ram : xbsIndex_r4/Single Port RAM  depth=16  initVector=0  distributed_mem=Block RAM  write_mode=Read Before Write  rst=off  init_reg=0  en=off  optimize_latency=off  latency=bram_latency  optimize=Area  dbl_ovrd=off  simulation_type=fast_sim  block_type=spram
  dout : Outport  VectorParamsAs1DForOutWhenUnconnected=off
  wires:
  ram/1 -> dout/1
  constant/1 -> ram/3
  din/1 -> ram/2
  counter/1 -> ram/1

== system rfsoc4x2_ospfb_128/pfb_fir_real7/pol1_in1_tap4/delay_bram ==
  din : Inport
  constant : xbsIndex_r4/Constant  const=1  gui_display_data_type=Fixed-point  arith_type=Boolean  n_bits=16  bin_pt=14  preci_type=Single  exp_width=8  frac_width=24  explicit_period=on  period=1  equ=P=C  opselect=C  inp2=PCIN>>17  opr=+  inp1=P  carry=CIN  dbl_ovrd=off  block_type=constant
  counter : xbsIndex_r4/Counter  cnt_type=Count Limited  cnt_to=DelayLen - bram_latency - 1  operation=Up  start_count=0  cnt_by_val=1  arith_type=Unsigned  n_bits=4  bin_pt=0  load_pin=off  rst=off  en=off  explicit_period=on  period=1  use_behavioral_HDL=on  implementation=Fabric  use_rpm=off  dbl_ovrd=off  block_type=counter
  ram : xbsIndex_r4/Single Port RAM  depth=16  initVector=0  distributed_mem=Block RAM  write_mode=Read Before Write  rst=off  init_reg=0  en=off  optimize_latency=off  latency=bram_latency  optimize=Area  dbl_ovrd=off  simulation_type=fast_sim  block_type=spram
  dout : Outport  VectorParamsAs1DForOutWhenUnconnected=off
  wires:
  ram/1 -> dout/1
  constant/1 -> ram/3
  din/1 -> ram/2
  counter/1 -> ram/1

== system rfsoc4x2_ospfb_128/pfb_fir_real7/pol1_in1_tap5/delay_bram ==
  din : Inport
  constant : xbsIndex_r4/Constant  const=1  gui_display_data_type=Fixed-point  arith_type=Boolean  n_bits=16  bin_pt=14  preci_type=Single  exp_width=8  frac_width=24  explicit_period=on  period=1  equ=P=C  opselect=C  inp2=PCIN>>17  opr=+  inp1=P  carry=CIN  dbl_ovrd=off  block_type=constant
  counter : xbsIndex_r4/Counter  cnt_type=Count Limited  cnt_to=DelayLen - bram_latency - 1  operation=Up  start_count=0  cnt_by_val=1  arith_type=Unsigned  n_bits=4  bin_pt=0  load_pin=off  rst=off  en=off  explicit_period=on  period=1  use_behavioral_HDL=on  implementation=Fabric  use_rpm=off  dbl_ovrd=off  block_type=counter
  ram : xbsIndex_r4/Single Port RAM  depth=16  initVector=0  distributed_mem=Block RAM  write_mode=Read Before Write  rst=off  init_reg=0  en=off  optimize_latency=off  latency=bram_latency  optimize=Area  dbl_ovrd=off  simulation_type=fast_sim  block_type=spram
  dout : Outport  VectorParamsAs1DForOutWhenUnconnected=off
  wires:
  ram/1 -> dout/1
  constant/1 -> ram/3
  din/1 -> ram/2
  counter/1 -> ram/1

== system rfsoc4x2_ospfb_128/pfb_fir_real7/pol1_in1_tap6/delay_bram ==
  din : Inport
  constant : xbsIndex_r4/Constant  const=1  gui_display_data_type=Fixed-point  arith_type=Boolean  n_bits=16  bin_pt=14  preci_type=Single  exp_width=8  frac_width=24  explicit_period=on  period=1  equ=P=C  opselect=C  inp2=PCIN>>17  opr=+  inp1=P  carry=CIN  dbl_ovrd=off  block_type=constant
  counter : xbsIndex_r4/Counter  cnt_type=Count Limited  cnt_to=DelayLen - bram_latency - 1  operation=Up  start_count=0  cnt_by_val=1  arith_type=Unsigned  n_bits=4  bin_pt=0  load_pin=off  rst=off  en=off  explicit_period=on  period=1  use_behavioral_HDL=on  implementation=Fabric  use_rpm=off  dbl_ovrd=off  block_type=counter
  ram : xbsIndex_r4/Single Port RAM  depth=16  initVector=0  distributed_mem=Block RAM  write_mode=Read Before Write  rst=off  init_reg=0  en=off  optimize_latency=off  latency=bram_latency  optimize=Area  dbl_ovrd=off  simulation_type=fast_sim  block_type=spram
  dout : Outport  VectorParamsAs1DForOutWhenUnconnected=off
  wires:
  ram/1 -> dout/1
  constant/1 -> ram/3
  din/1 -> ram/2
  counter/1 -> ram/1

== system rfsoc4x2_ospfb_128/pfb_fir_real7/pol1_in1_tap7/delay_bram ==
  din : Inport
  constant : xbsIndex_r4/Constant  const=1  gui_display_data_type=Fixed-point  arith_type=Boolean  n_bits=16  bin_pt=14  preci_type=Single  exp_width=8  frac_width=24  explicit_period=on  period=1  equ=P=C  opselect=C  inp2=PCIN>>17  opr=+  inp1=P  carry=CIN  dbl_ovrd=off  block_type=constant
  counter : xbsIndex_r4/Counter  cnt_type=Count Limited  cnt_to=DelayLen - bram_latency - 1  operation=Up  start_count=0  cnt_by_val=1  arith_type=Unsigned  n_bits=4  bin_pt=0  load_pin=off  rst=off  en=off  explicit_period=on  period=1  use_behavioral_HDL=on  implementation=Fabric  use_rpm=off  dbl_ovrd=off  block_type=counter
  ram : xbsIndex_r4/Single Port RAM  depth=16  initVector=0  distributed_mem=Block RAM  write_mode=Read Before Write  rst=off  init_reg=0  en=off  optimize_latency=off  latency=bram_latency  optimize=Area  dbl_ovrd=off  simulation_type=fast_sim  block_type=spram
  dout : Outport  VectorParamsAs1DForOutWhenUnconnected=off
  wires:
  ram/1 -> dout/1
  constant/1 -> ram/3
  din/1 -> ram/2
  counter/1 -> ram/1

== system rfsoc4x2_ospfb_128/pfb_fir_real7/pol1_in1_tap8/delay_bram ==
  din : Inport
  constant : xbsIndex_r4/Constant  const=1  gui_display_data_type=Fixed-point  arith_type=Boolean  n_bits=16  bin_pt=14  preci_type=Single  exp_width=8  frac_width=24  explicit_period=on  period=1  equ=P=C  opselect=C  inp2=PCIN>>17  opr=+  inp1=P  carry=CIN  dbl_ovrd=off  block_type=constant
  counter : xbsIndex_r4/Counter  cnt_type=Count Limited  cnt_to=DelayLen - bram_latency - 1  operation=Up  start_count=0  cnt_by_val=1  arith_type=Unsigned  n_bits=4  bin_pt=0  load_pin=off  rst=off  en=off  explicit_period=on  period=1  use_behavioral_HDL=on  implementation=Fabric  use_rpm=off  dbl_ovrd=off  block_type=counter
  ram : xbsIndex_r4/Single Port RAM  depth=16  initVector=0  distributed_mem=Block RAM  write_mode=Read Before Write  rst=off  init_reg=0  en=off  optimize_latency=off  latency=bram_latency  optimize=Area  dbl_ovrd=off  simulation_type=fast_sim  block_type=spram
  dout : Outport  VectorParamsAs1DForOutWhenUnconnected=off
  wires:
  ram/1 -> dout/1
  constant/1 -> ram/3
  din/1 -> ram/2
  counter/1 -> ram/1

== system rfsoc4x2_ospfb_128/pfb_fir_real7/pol1_in1_tap9/delay_bram ==
  din : Inport
  constant : xbsIndex_r4/Constant  const=1  gui_display_data_type=Fixed-point  arith_type=Boolean  n_bits=16  bin_pt=14  preci_type=Single  exp_width=8  frac_width=24  explicit_period=on  period=1  equ=P=C  opselect=C  inp2=PCIN>>17  opr=+  inp1=P  carry=CIN  dbl_ovrd=off  block_type=constant
  counter : xbsIndex_r4/Counter  cnt_type=Count Limited  cnt_to=DelayLen - bram_latency - 1  operation=Up  start_count=0  cnt_by_val=1  arith_type=Unsigned  n_bits=4  bin_pt=0  load_pin=off  rst=off  en=off  explicit_period=on  period=1  use_behavioral_HDL=on  implementation=Fabric  use_rpm=off  dbl_ovrd=off  block_type=counter
  ram : xbsIndex_r4/Single Port RAM  depth=16  initVector=0  distributed_mem=Block RAM  write_mode=Read Before Write  rst=off  init_reg=0  en=off  optimize_latency=off  latency=bram_latency  optimize=Area  dbl_ovrd=off  simulation_type=fast_sim  block_type=spram
  dout : Outport  VectorParamsAs1DForOutWhenUnconnected=off
  wires:
  ram/1 -> dout/1
  constant/1 -> ram/3
  din/1 -> ram/2
  counter/1 -> ram/1

== system rfsoc4x2_ospfb_128/q1/munge_in/join ==
  in1 : Inport
  in2 : Inport  Port=2
  concatenate : xbsIndex_r4/Concat  num_inputs=2  dbl_ovrd=off  block_type=concat
  reinterpret1 : xbsIndex_r4/Reinterpret  force_arith_type=on  arith_type=Unsigned  force_bin_pt=on  bin_pt=0  block_type=reinterpret
      settings: infoedit="Changes signal type without altering the binary representation.   You can changed the signal between signed and unsigned, and relocate the binary point.<br><br>Hardware notes: In hardware this block costs nothing.<br><br>Example:  Suppose the input is 6 bits wide, signed, with 2 fractional bits, and the output is forced to unsigned with 0 fractional bits.  Then an input of -2.0 (1110.00 in binary 2's complement) becomes an output of 56 (111000 in binary)."
  reinterpret2 : xbsIndex_r4/Reinterpret  force_arith_type=on  arith_type=Unsigned  force_bin_pt=on  bin_pt=0  block_type=reinterpret
      settings: infoedit="Changes signal type without altering the binary representation.   You can changed the signal between signed and unsigned, and relocate the binary point.<br><br>Hardware notes: In hardware this block costs nothing.<br><br>Example:  Suppose the input is 6 bits wide, signed, with 2 fractional bits, and the output is forced to unsigned with 0 fractional bits.  Then an input of -2.0 (1110.00 in binary 2's complement) becomes an output of 56 (111000 in binary)."
  bus_out : Outport  VectorParamsAs1DForOutWhenUnconnected=off
  wires:
  reinterpret2/1 -> concatenate/2
  in2/1 -> reinterpret2/1
  reinterpret1/1 -> concatenate/1
  in1/1 -> reinterpret1/1
  concatenate/1 -> bus_out/1

== system rfsoc4x2_ospfb_128/q1/munge_in/split ==
  bus_in : Inport
  reinterpret1 : xbsIndex_r4/Reinterpret  force_arith_type=on  arith_type=Unsigned  force_bin_pt=on  bin_pt=0  block_type=reinterpret
  reinterpret2 : xbsIndex_r4/Reinterpret  force_arith_type=on  arith_type=Unsigned  force_bin_pt=on  bin_pt=0  block_type=reinterpret
  slice1 : xbsIndex_r4/Slice  nbits=32  boolean_output=off  mode=Upper Bit Location + Width  bit1=-32  base1=MSB of Input  bit0=0  base0=LSB of Input  dbl_ovrd=off  block_type=slice
  slice2 : xbsIndex_r4/Slice  nbits=32  boolean_output=off  mode=Upper Bit Location + Width  bit1=0  base1=MSB of Input  bit0=0  base0=LSB of Input  dbl_ovrd=off  block_type=slice
  msb_out2 : Outport  VectorParamsAs1DForOutWhenUnconnected=off
  lsb_out1 : Outport  Port=2  VectorParamsAs1DForOutWhenUnconnected=off
  wires:
  reinterpret1/1 -> lsb_out1/1
  slice1/1 -> reinterpret1/1
  reinterpret2/1 -> msb_out2/1
  slice2/1 -> reinterpret2/1
  bus_in/1 -> slice1/1, slice2/1

== system rfsoc4x2_ospfb_128/q1/munge_out/join ==
  in1 : Inport
  in2 : Inport  Port=2
  concatenate : xbsIndex_r4/Concat  num_inputs=2  dbl_ovrd=off  block_type=concat
  reinterpret1 : xbsIndex_r4/Reinterpret  force_arith_type=on  arith_type=Unsigned  force_bin_pt=on  bin_pt=0  block_type=reinterpret
      settings: infoedit="Changes signal type without altering the binary representation.   You can changed the signal between signed and unsigned, and relocate the binary point.<br><br>Hardware notes: In hardware this block costs nothing.<br><br>Example:  Suppose the input is 6 bits wide, signed, with 2 fractional bits, and the output is forced to unsigned with 0 fractional bits.  Then an input of -2.0 (1110.00 in binary 2's complement) becomes an output of 56 (111000 in binary)."
  reinterpret2 : xbsIndex_r4/Reinterpret  force_arith_type=on  arith_type=Unsigned  force_bin_pt=on  bin_pt=0  block_type=reinterpret
      settings: infoedit="Changes signal type without altering the binary representation.   You can changed the signal between signed and unsigned, and relocate the binary point.<br><br>Hardware notes: In hardware this block costs nothing.<br><br>Example:  Suppose the input is 6 bits wide, signed, with 2 fractional bits, and the output is forced to unsigned with 0 fractional bits.  Then an input of -2.0 (1110.00 in binary 2's complement) becomes an output of 56 (111000 in binary)."
  bus_out : Outport  VectorParamsAs1DForOutWhenUnconnected=off
  wires:
  reinterpret2/1 -> concatenate/2
  in2/1 -> reinterpret2/1
  reinterpret1/1 -> concatenate/1
  in1/1 -> reinterpret1/1
  concatenate/1 -> bus_out/1
